simulink model "sistemaP3"  (R2023a)
settings: Solver=ode15s  StartTime=0.0  StopTime=10  MaxStep=1E-2  RelTol=1e-3
libraries: fl_lib x14, nesl_utility x8, slpidlib x1
settings Model: LastModifiedBy=vayam
settings DataIOCC: SaveFormat=Array  SaveOutput=off  SignalLogging=off  DSMLogging=off  ReturnWorkspaceOutputs=off  TimeSaveName=t
settings DebuggingCC: AlgebraicLoopMsg=none  ArtificialAlgebraicLoopMsg=none  MaxConsecutiveZCsMsg=none  ModelReferenceExtraNoncontSigs=none  OperatingPointInterfaceChecksumMismatchMsg=none
settings ModelReferenceCC: UpdateModelReferenceTargets=IfOutOfDate
settings RTWCC: GPUComputeCapability=5.0

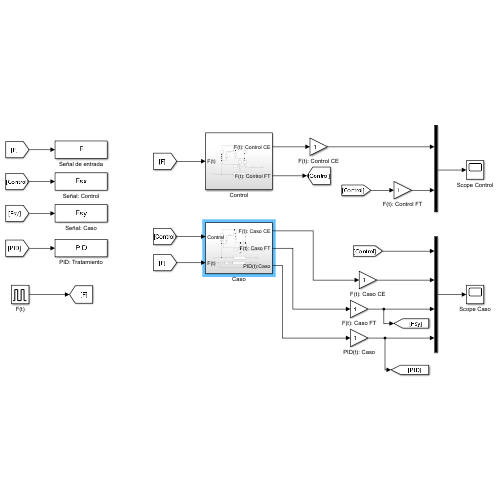
[thumbnail: Simulink's stored preview of the top-level diagram]
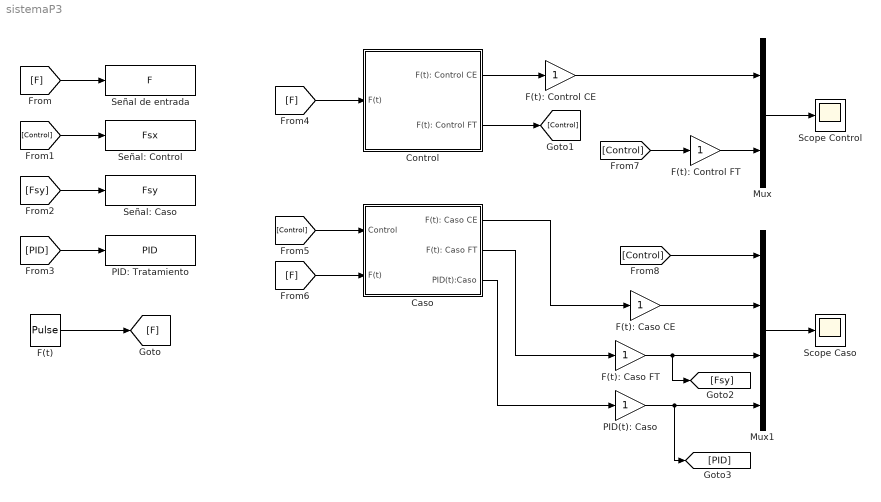
== system sistemaP3 ==
  Caso : Subsystem
  Control : Subsystem
  F(t) : DiscretePulseGenerator  PulseType=Time based  Period=10  PulseWidth=10  PhaseDelay=1
  F(t): Caso CE : Gain
  F(t): Caso FT : Gain
  F(t): Control CE : Gain
  F(t): Control FT : Gain
  Mux : Mux  Inputs=2
  Mux1 : Mux
  PID(t): Caso : Gain
  PID: Tratamiento : ToWorkspace  VariableName=PID  SampleTime=-1
  Scope Caso : Scope
  Scope Control : Scope
  Señal de entrada : ToWorkspace  VariableName=F  SampleTime=-1
  Señal: Caso : ToWorkspace  VariableName=Fsy  SampleTime=-1
  Señal: Control : ToWorkspace  VariableName=Fsx  SampleTime=-1
  wires:
  [PID] -> PID: Tratamiento/1
  [Fsy] -> Señal: Caso/1
  [Control] -> Señal: Control/1
  [F] -> Señal de entrada/1
  F(t)/1 -> [F]
  [F] -> Control/1(F(t))
  [Control] -> Caso/1(Control)
  [F] -> Caso/2(F(t))
  Control/1(F(t): Control CE) -> F(t): Control CE/1
  Control/2(F(t): Control FT) -> [Control]
  F(t): Control CE/1 -> Mux/1
  Mux/1 -> Scope Control/1
  [Control] -> F(t): Control FT/1
  F(t): Control FT/1 -> Mux/2
  F(t): Caso CE/1 -> Mux1/2
  Caso/1(F(t): Caso CE) -> F(t): Caso CE/1
  Caso/2(F(t): Caso FT) -> F(t): Caso FT/1
  F(t): Caso FT/1 -> [Fsy], Mux1/3
  Caso/3(PID(t):Caso) -> PID(t): Caso/1
  PID(t): Caso/1 -> [PID], Mux1/4
  [Control] -> Mux1/1
  Mux1/1 -> Scope Caso/1

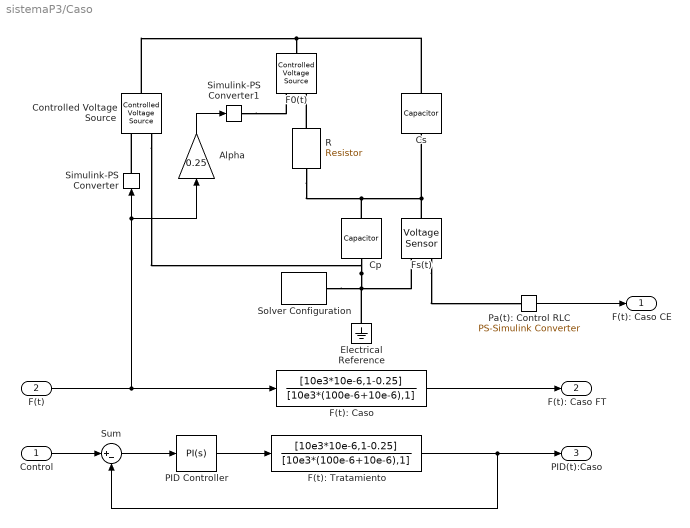
== system sistemaP3/Caso ==
  Control : Inport
  F(t) : Inport  Port=2
  Alpha : Gain  Gain=0.25
  Controlled Voltage Source : fl_lib/Electrical/Electrical Sources/Controlled Voltage Source
  Cp : fl_lib/Electrical/Electrical Elements/Capacitor  c=100e-6 F  r=1e-6 Ohm  g=0 1/Ohm  i_specify=off  i_priority=None  i=0 A  i_nominal_specify=off  i_nominal_unit=A  i_nominal_value=1  v_specify=off  v_priority=None  v=0 V  v_nominal_specify=off  v_nominal_unit=V  v_nominal_value=1  vc_specify=off  vc_priority=High  vc=0 V  vc_nominal_specify=off  vc_nominal_unit=V  vc_nominal_value=1
  Cs : fl_lib/Electrical/Electrical Elements/Capacitor  c=10e-6 F  r=1e-6 Ohm  g=0 1/Ohm  i_specify=off  i_priority=None  i=0 A  i_nominal_specify=off  i_nominal_unit=A  i_nominal_value=1  v_specify=off  v_priority=None  v=0 V  v_nominal_specify=off  v_nominal_unit=V  v_nominal_value=1  vc_specify=off  vc_priority=High  vc=0 V  vc_nominal_specify=off  vc_nominal_unit=V  vc_nominal_value=1
  Electrical Reference : fl_lib/Electrical/Electrical Elements/Electrical Reference
  F(t): Caso : TransferFcn  Numerator=[10e3*10e-6,1-0.25]  Denominator=[10e3*(100e-6+10e-6),1]
  F(t): Tratamiento : TransferFcn  Numerator=[10e3*10e-6,1-0.25]  Denominator=[10e3*(100e-6+10e-6),1]
  F0(t) : fl_lib/Electrical/Electrical Sources/Controlled Voltage Source
  Fs(t) : fl_lib/Electrical/Electrical Sensors/Voltage Sensor
  PID Controller : slpidlib/PID Controller  Controller=PI  Form=Parallel  TimeDomain=Continuous-time  UseExternalTs=off  SampleTime=-1  IntegratorMethod=Forward Euler  FilterMethod=Forward Euler  ControllerParametersSource=internal  P=0.217389946339663  I=3665.03624206912  UseKiTs=off  D=0  N=100  UseFilter=on  TunerSelectOption=Transfer Function Based (PID Tuner App)  InitialConditionSource=internal  InitialConditionForIntegrator=0  InitialConditionForFilter=0  DifferentiatorICPrevScaledInput=0  ExternalReset=none  TrackingMode=off  Kt=1  LimitOutput=off  SatLimitsSource=internal  UpperSaturationLimit=inf  LowerSaturationLimit=-inf  LinearizeAsGain=on  AntiWindupMode=none  Kb=1  LimitIntegrator=off  UpperIntegratorSaturationLimit=inf  LowerIntegratorSaturationLimit=-inf  POutMin=[]  POutMax=[]  IOutMin=[]  IOutMax=[]  DOutMin=[]  DOutMax=[]  NOutMin=[]  NOutMax=[]  SumOutMin=[]  SumOutMax=[]  SaturationOutMin=[]  SaturationOutMax=[]  PParamMin=[]  PParamMax=[]  IParamMin=[]  IParamMax=[]  DParamMin=[]  DParamMax=[]  NParamMin=[]  NParamMax=[]  KbParamMin=[]  KbParamMax=[]  KtParamMin=[]  KtParamMax=[]  KbOutMin=[]  KbOutMax=[]  KtOutMin=[]  KtOutMax=[]  IntegratorOutMin=[]  IntegratorOutMax=[]  FilterOutMin=[]  FilterOutMax=[]  SumI1OutMin=[]  SumI1OutMax=[]  SumI2OutMin=[]  SumI2OutMax=[]  SumI3OutMin=[]  SumI3OutMax=[]  SumI4OutMin=[]  SumI4OutMax=[]  SumDOutMin=[]  SumDOutMax=[]  DifferentiatorOutMin=[]  DifferentiatorOutMax=[]  FilterDiffOutCoefMin=[]  FilterDiffOutCoefMax=[]  ReciprocalOutMin=[]  ReciprocalOutMax=[]  SumDenOutMin=[]  SumDenOutMax=[]  SumNumOutMin=[]  SumNumOutMax=[]  DivideOutMin=[]  DivideOutMax=[]  UdiffTsProdOutMin=[]  UdiffTsProdOutMax=[]  NTsProdOutMin=[]  NTsProdOutMax=[]  UintegralTsProdOutMin=[]  UintegralTsProdOutMax=[]  UngainTsProdOutMin=[]  UngainTsProdOutMax=[]  ClampingZeroOutDataTypeStr=Inherit: Inherit via back propagation  ClampingZeroOutMin=[]  ClampingZeroOutMax=[]  FilterDenConstantOutDataTypeStr=Inherit: Inherit via back propagation  FilterDenConstantOutMin=[]  FilterDenConstantOutMax=[]  PCopyOutDataTypeStr=Inherit: Inherit via back propagation  PCopyOutMin=[]  PCopyOutMax=[]  NCopyOutDataTypeStr=Inherit: Inherit via back propagation  NCopyOutMin=[]  NCopyOutMax=[]  IntegratorContinuousStateAttributes=''  IntegratorStateMustResolveToSignalObject=off  IntegratorRTWStateStorageClass=Auto  FilterContinuousStateAttributes=''  FilterStateMustResolveToSignalObject=off  FilterRTWStateStorageClass=Auto  ParallelPVariant=InternalParameters  IdealPVariant=Disabled  IVariant=InternalParameters  DVariant=Disabled  IntegratorVariant=Continuous  SatVariant=Disabled  AWVariant=Passthrough  PCopyVariant=Disabled  TRVariant=Disabled  FdbkBlocksVariant=Forward  IdealPFdbkVariant=Disabled  SatFdbkVariant=Disabled  DerivativeFilterVariant=Disabled  NVariant=Disabled  NCopyVariant=Disabled_SignalSpec  FilterICVariant=Disabled  IntegratorICVariant=InternalICs  ExternalResetVariant=Disabled  TRSumVariant=Passthrough  SumFdbkVariant=Disabled  SumVariant=Sum_PI  TsampFilterVariant=InternalTs  TsampNgainVariant=Passthrough  TsampIntegralVariant=Disabled_SignalSpec  ExternalSaturationOutDataTypeStr=Inherit: Same as second input
  Pa(t): Control RLC : nesl_utility/PS-Simulink Converter  PhysicalDomain=network_engine_domain  SubClassName=ps_output  LeftPortType=input  RightPortType=output  PseudoPeriodic=off  Frequencies=[]  VectorFormat=inherit  Unit=inherit  AffineConversion=off
  R : fl_lib/Electrical/Electrical Elements/Resistor  R=10e3 Ohm  i_specify=off  i_priority=None  i=0 A  i_nominal_specify=off  i_nominal_unit=A  i_nominal_value=1  v_specify=off  v_priority=None  v=0 V  v_nominal_specify=off  v_nominal_unit=V  v_nominal_value=1
  Simulink-PS Converter : nesl_utility/Simulink-PS Converter  PhysicalDomain=network_engine_domain  SubClassName=ps_input  LeftPortType=input  RightPortType=output  PseudoPeriodic=off  Frequencies=[]  NoiseDistribution=none  NoiseParameters=[]  Unit=1  AffineConversion=off  FilteringAndDerivatives=provide  SimscapeFilterOrder=1  InputFilterTimeConstant=0.001  UdotUserProvided=0
  Simulink-PS Converter1 : nesl_utility/Simulink-PS Converter  PhysicalDomain=network_engine_domain  SubClassName=ps_input  LeftPortType=input  RightPortType=output  PseudoPeriodic=off  Frequencies=[]  NoiseDistribution=none  NoiseParameters=[]  Unit=1  AffineConversion=off  FilteringAndDerivatives=provide  SimscapeFilterOrder=1  InputFilterTimeConstant=0.001  UdotUserProvided=0
  Solver Configuration : nesl_utility/Solver Configuration  PhysicalDomain=network_engine_domain  SubClassName=solver  LeftPortType=input  RightPortType=generic  Tones=[]  Harmonics=[]  SimulateNoise=off  Profile=off  UseLocalSampling=off  EnableSwitchedLinearOptims=on  FrequencyDomain=off  UseCCode=off  RelTol=0.001  AbsTol=0.001  MinStep=1e-09  ToWorkspace=off  RevertToSquareIcSolve=off  NumHomotopyIterations=100  PhasorMode=off  PhasorModeNumHarmonics=1  ConsistencySolver=NEWTON_XTOL_AFTER_FTOL  IndexReductionMethod=DerivativeReplacement  DoDC=off  ResidualTolerance=1e-09  ConsistencyTolSource=GLOBAL  ConsistencyAbsTol=0.001  ConsistencyRelTol=0.001  ConsistencyTolFactor=0.001  UseLocalSolver=off  LocalSolverChoice=NE_BACKWARD_EULER_ADVANCER  ResolveIndetEquations=on  FunctionEvalNumThread=1  LocalSolverSampleTime=0.001  DoFixedCost=off  MaxNonlinIter=3  MaxModeIter=2  ComputeImpulses=off  ImpulseIterations=2  LinearAlgebra=auto  LinearAlgebraNumThread=0  EquationFormulation=NE_TIME_EF  DelaysMemoryBudget=1024  AutomaticFiltering=on  FilteringTimeConstant=0.001  PartitionStorageMethod=AS_NEEDED  PartitionMemoryBudget=1024  PartitionMethod=ROBUST
  Sum : Sum  Inputs=|+-
  F(t): Caso CE : Outport
  F(t): Caso FT : Outport  Port=2
  PID(t):Caso : Outport  Port=3
  wires:
  F(t)/1 -> Alpha/1, Simulink-PS Converter/1, F(t): Caso/1
  F(t): Caso/1 -> F(t): Caso FT/1
  Alpha/1 -> Simulink-PS Converter1/1
  Pa(t): Control RLC/1 -> F(t): Caso CE/1
  Control/1 -> Sum/1
  Sum/1 -> PID Controller/1
  PID Controller/1 -> F(t): Tratamiento/1
  F(t): Tratamiento/1 -> Sum/2, PID(t):Caso/1
  connections:
  Simulink-PS Converter/RConn1 -- Controlled Voltage Source/RConn1
  R/LConn1 -- F0(t)/RConn2
  Simulink-PS Converter1/RConn1 -- F0(t)/RConn1
  Controlled Voltage Source/LConn1 -- F0(t)/LConn1 -- Cs/LConn1
  Cs/RConn1 -- Fs(t)/LConn1 -- R/RConn1 -- Cp/LConn1
  Fs(t)/RConn2 -- Electrical Reference/LConn1 -- Solver Configuration/RConn1 -- Cp/RConn1 -- Controlled Voltage Source/RConn2
  Fs(t)/RConn1 -- Pa(t): Control RLC/LConn1

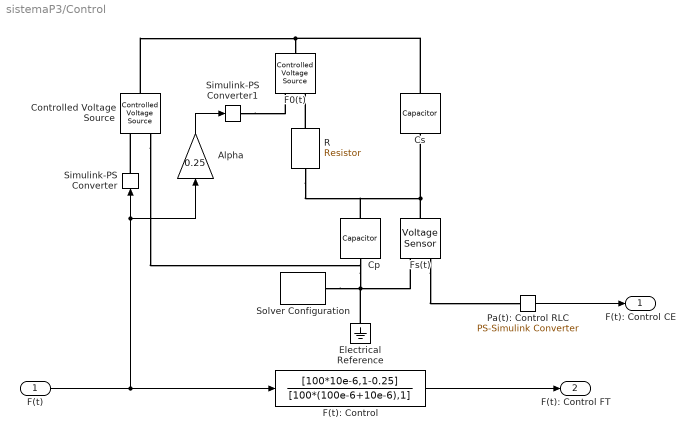
== system sistemaP3/Control ==
  F(t) : Inport
  Alpha : Gain  Gain=0.25
  Controlled Voltage Source : fl_lib/Electrical/Electrical Sources/Controlled Voltage Source
  Cp : fl_lib/Electrical/Electrical Elements/Capacitor  c=100e-6 F  r=1e-6 Ohm  g=0 1/Ohm  i_specify=off  i_priority=None  i=0 A  i_nominal_specify=off  i_nominal_unit=A  i_nominal_value=1  v_specify=off  v_priority=None  v=0 V  v_nominal_specify=off  v_nominal_unit=V  v_nominal_value=1  vc_specify=off  vc_priority=High  vc=0 V  vc_nominal_specify=off  vc_nominal_unit=V  vc_nominal_value=1
  Cs : fl_lib/Electrical/Electrical Elements/Capacitor  c=10e-6 F  r=1e-6 Ohm  g=0 1/Ohm  i_specify=off  i_priority=None  i=0 A  i_nominal_specify=off  i_nominal_unit=A  i_nominal_value=1  v_specify=off  v_priority=None  v=0 V  v_nominal_specify=off  v_nominal_unit=V  v_nominal_value=1  vc_specify=off  vc_priority=High  vc=0 V  vc_nominal_specify=off  vc_nominal_unit=V  vc_nominal_value=1
  Electrical Reference : fl_lib/Electrical/Electrical Elements/Electrical Reference
  F(t): Control : TransferFcn  Numerator=[100*10e-6,1-0.25]  Denominator=[100*(100e-6+10e-6),1]
  F0(t) : fl_lib/Electrical/Electrical Sources/Controlled Voltage Source
  Fs(t) : fl_lib/Electrical/Electrical Sensors/Voltage Sensor
  Pa(t): Control RLC : nesl_utility/PS-Simulink Converter  PhysicalDomain=network_engine_domain  SubClassName=ps_output  LeftPortType=input  RightPortType=output  PseudoPeriodic=off  Frequencies=[]  VectorFormat=inherit  Unit=inherit  AffineConversion=off
  R : fl_lib/Electrical/Electrical Elements/Resistor  R=100 Ohm  i_specify=off  i_priority=None  i=0 A  i_nominal_specify=off  i_nominal_unit=A  i_nominal_value=1  v_specify=off  v_priority=None  v=0 V  v_nominal_specify=off  v_nominal_unit=V  v_nominal_value=1
  Simulink-PS Converter : nesl_utility/Simulink-PS Converter  PhysicalDomain=network_engine_domain  SubClassName=ps_input  LeftPortType=input  RightPortType=output  PseudoPeriodic=off  Frequencies=[]  NoiseDistribution=none  NoiseParameters=[]  Unit=1  AffineConversion=off  FilteringAndDerivatives=provide  SimscapeFilterOrder=1  InputFilterTimeConstant=0.001  UdotUserProvided=0
  Simulink-PS Converter1 : nesl_utility/Simulink-PS Converter  PhysicalDomain=network_engine_domain  SubClassName=ps_input  LeftPortType=input  RightPortType=output  PseudoPeriodic=off  Frequencies=[]  NoiseDistribution=none  NoiseParameters=[]  Unit=1  AffineConversion=off  FilteringAndDerivatives=provide  SimscapeFilterOrder=1  InputFilterTimeConstant=0.001  UdotUserProvided=0
  Solver Configuration : nesl_utility/Solver Configuration  PhysicalDomain=network_engine_domain  SubClassName=solver  LeftPortType=input  RightPortType=generic  Tones=[]  Harmonics=[]  SimulateNoise=off  Profile=off  UseLocalSampling=off  EnableSwitchedLinearOptims=on  FrequencyDomain=off  UseCCode=off  RelTol=0.001  AbsTol=0.001  MinStep=1e-09  ToWorkspace=off  RevertToSquareIcSolve=off  NumHomotopyIterations=100  PhasorMode=off  PhasorModeNumHarmonics=1  ConsistencySolver=NEWTON_XTOL_AFTER_FTOL  IndexReductionMethod=DerivativeReplacement  DoDC=off  ResidualTolerance=1e-09  ConsistencyTolSource=GLOBAL  ConsistencyAbsTol=0.001  ConsistencyRelTol=0.001  ConsistencyTolFactor=0.001  UseLocalSolver=off  LocalSolverChoice=NE_BACKWARD_EULER_ADVANCER  ResolveIndetEquations=on  FunctionEvalNumThread=1  LocalSolverSampleTime=0.001  DoFixedCost=off  MaxNonlinIter=3  MaxModeIter=2  ComputeImpulses=off  ImpulseIterations=2  LinearAlgebra=auto  LinearAlgebraNumThread=0  EquationFormulation=NE_TIME_EF  DelaysMemoryBudget=1024  AutomaticFiltering=on  FilteringTimeConstant=0.001  PartitionStorageMethod=AS_NEEDED  PartitionMemoryBudget=1024  PartitionMethod=ROBUST
  F(t): Control CE : Outport
  F(t): Control FT : Outport  Port=2
  wires:
  F(t)/1 -> Alpha/1, Simulink-PS Converter/1, F(t): Control/1
  F(t): Control/1 -> F(t): Control FT/1
  Alpha/1 -> Simulink-PS Converter1/1
  Pa(t): Control RLC/1 -> F(t): Control CE/1
  connections:
  Simulink-PS Converter/RConn1 -- Controlled Voltage Source/RConn1
  R/LConn1 -- F0(t)/RConn2
  Simulink-PS Converter1/RConn1 -- F0(t)/RConn1
  Controlled Voltage Source/LConn1 -- Cs/LConn1 -- F0(t)/LConn1
  Fs(t)/LConn1 -- Cp/LConn1 -- R/RConn1 -- Cs/RConn1
  Solver Configuration/RConn1 -- Controlled Voltage Source/RConn2 -- Cp/RConn1 -- Fs(t)/RConn2 -- Electrical Reference/LConn1
  Fs(t)/RConn1 -- Pa(t): Control RLC/LConn1
